simulink model "cmdvectPmsm (1)"  (R2023b)
settings: Solver=FixedStepAuto  StartTime=0.0  StopTime=0.6  FixedStep=1e-5  MaxStep=1e-6  RelTol=1e-6
undefined symbols (not defined in the file): A1, A2, B1, B2, fs, J, Ld, Lq, P, Phif
libraries: spsTriangleGeneratorLib x1
settings Model: Creator=HP  LastModifiedBy=HP
settings SolverCC: ZeroCrossAlgorithm=Adaptive
settings DebuggingCC: IgnoredZcDiagnostic=none

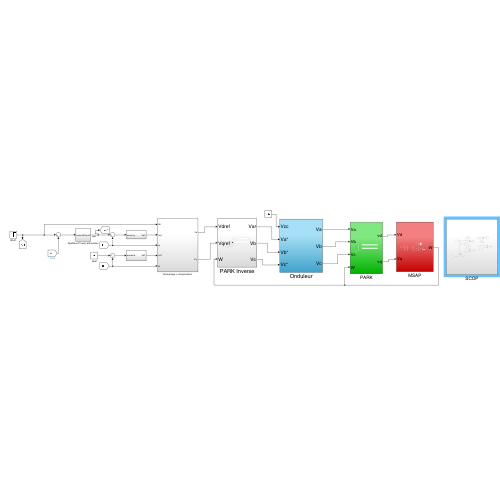
[thumbnail: Simulink's stored preview of the top-level diagram]
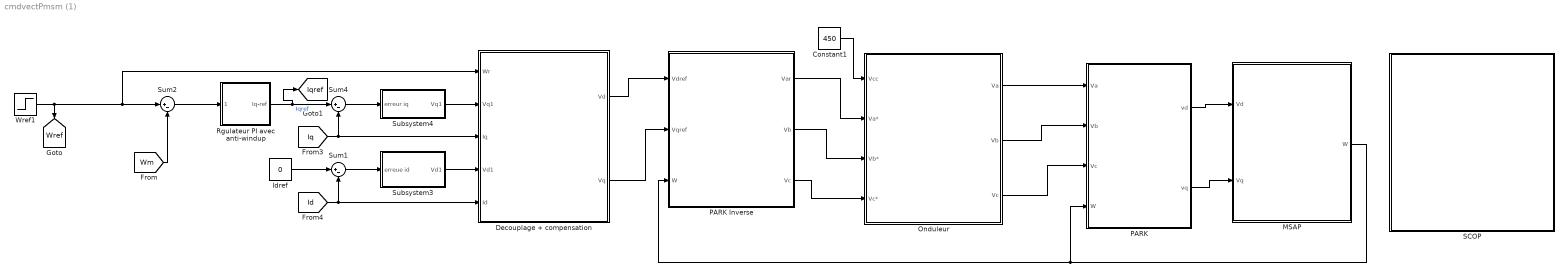
== system cmdvectPmsm (1) ==
  " Idref" : Constant  Value=0
  Constant1 : Constant  Value=450
  "Decouplage + compensation " : Subsystem
  MSAP : Subsystem
  Onduleur : Subsystem
  PARK : Subsystem
  PARK Inverse : Subsystem
  Rgulateur PI avec anti-windup : Subsystem
  SCOP : Subsystem
  Subsystem3 : Subsystem
  Subsystem4 : Subsystem
  Sum1 : Sum  Inputs=|+-
  Sum2 : Sum  Inputs=|+-
  Sum4 : Sum  Inputs=|+-
  Wref1 : Step  Time=0.3  Before=500  After=1000  SampleTime=0
  tag scope: Iqref=global, Wref=global
  wires:
  PARK/1(vd) -> MSAP/1(Vd)
  PARK/2(vq) -> MSAP/2(Vq)
  "Decouplage + compensation "/2("Vq ") -> PARK Inverse/2(Vqref)
  "Decouplage + compensation "/1(Vd) -> PARK Inverse/1(Vdref)
  Subsystem4/1(Vq1) -> "Decouplage + compensation "/2("Vq1 ")
  Subsystem3/1(Vd1) -> "Decouplage + compensation "/4("Vd1 ")
  [Iq] -> Sum4/2, "Decouplage + compensation "/3(Iq)
  Rgulateur PI avec anti-windup/1(Iq-ref) -> [Iqref], Sum4/1  "Iqref"
  Sum4/1 -> Subsystem4/1(erreur iq)
  [Id] -> "Decouplage + compensation "/5(Id), Sum1/2
  Sum1/1 -> Subsystem3/1(erreue id)
  MSAP/1(W) -> PARK Inverse/3(W), PARK/4(W)
  Wref1/1 -> [Wref], "Decouplage + compensation "/1("Wr "), Sum2/1
  " Idref"/1 -> Sum1/1
  Sum2/1 -> Rgulateur PI avec anti-windup/1(erreur Wr)
  Onduleur/1(Va) -> PARK/1(Va)
  Onduleur/2(Vb) -> PARK/2(Vb)
  Onduleur/3(Vc) -> PARK/3(Vc)
  PARK Inverse/1(Var) -> Onduleur/2(Va*)
  PARK Inverse/2(Vb) -> Onduleur/3(Vb*)
  PARK Inverse/3(Vc) -> Onduleur/4(Vc*)
  Constant1/1 -> Onduleur/1(Vcc)
  [Wm] -> Sum2/2

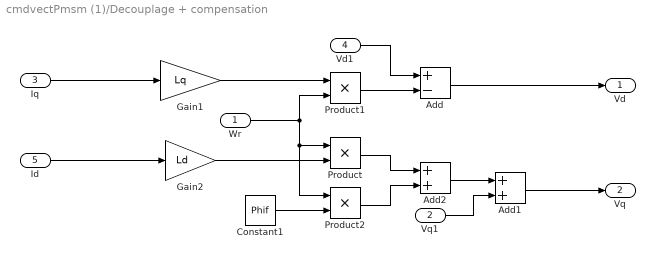
== system cmdvectPmsm (1)/Decouplage + compensation  ==
  "Wr " : Inport
  "Vq1 " : Inport  Port=2
  Iq : Inport  Port=3
  "Vd1 " : Inport  Port=4
  Id : Inport  Port=5
  Add : Sum  Inputs=+-
  Add1 : Sum
  Add2 : Sum
  Constant1 : Constant  Value=Phif
  Gain1 : Gain  Gain=Lq
  Gain2 : Gain  Gain=Ld
  Product : Product
  Product1 : Product
  Product2 : Product
  Vd : Outport
  "Vq " : Outport  Port=2
  wires:
  Iq/1 -> Gain1/1
  Add2/1 -> Add1/1
  Product1/1 -> Add/2
  Add1/1 -> "Vq "/1
  Add/1 -> Vd/1
  Product/1 -> Add2/1
  Product2/1 -> Add2/2
  Gain2/1 -> Product/2
  "Vd1 "/1 -> Add/1
  "Wr "/1 -> Product2/1, Product/1, Product1/2
  Gain1/1 -> Product1/1
  "Vq1 "/1 -> Add1/2
  Id/1 -> Gain2/1
  Constant1/1 -> Product2/2

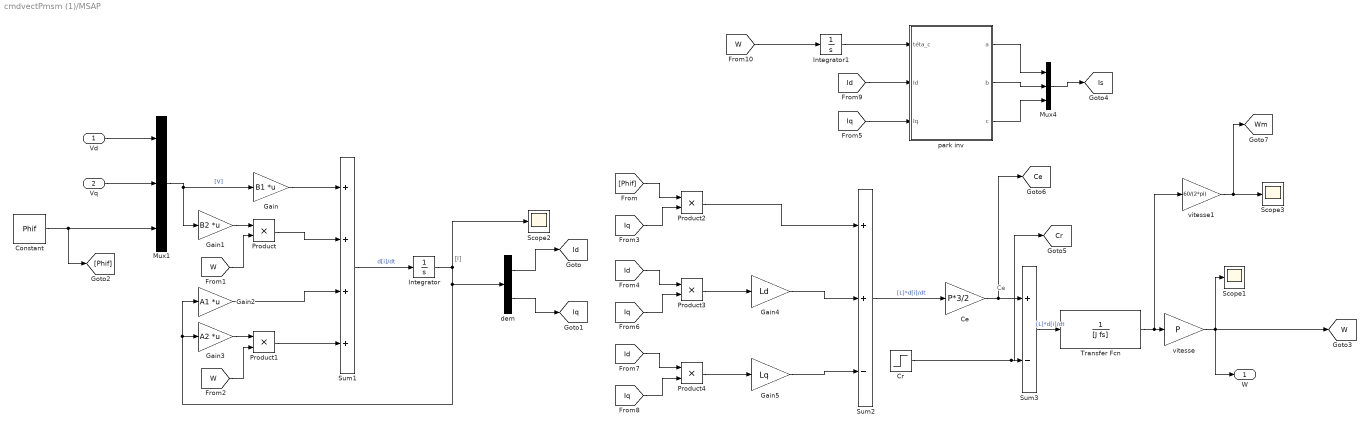
== system cmdvectPmsm (1)/MSAP ==
  note: Ce
  note: [I]
  Vd : Inport
  Vq : Inport  Port=2
  Ce : Gain  Gain=P*3/2
  Constant : Constant  Value=Phif
  Cr : Step  Time=0.3  Before=0.5  After=10  SampleTime=0
  Gain : Gain  Gain=B1  Multiplication=Matrix(K*u)
  Gain1 : Gain  Gain=B2  Multiplication=Matrix(K*u)
  Gain2 : Gain  Gain=A1  Multiplication=Matrix(K*u)
  Gain3 : Gain  Gain=A2  Multiplication=Matrix(K*u)
  Gain4 : Gain  Gain=Ld
  Gain5 : Gain  Gain=Lq
  Integrator : Integrator
  Integrator1 : Integrator
  Mux1 : Mux  Inputs=3
  Mux4 : Mux  Inputs=3
  Product{,1..4} (5 alike) : Product
  Scope1 : Scope
  Scope2 : Scope
  Scope3 : Scope
  Sum1 : Sum  Inputs=++++
  Sum2 : Sum  Inputs=++-
  Sum3 : Sum  Inputs=+-
  Transfer Fcn : TransferFcn  Denominator=[J fs]
  dem : Demux  Outputs=2
  park inv : Subsystem
  vitesse : Gain  Gain=P
  vitesse1 : Gain  Gain=60/(2*pi)
  W : Outport
  tag scope: Ce=global, Cr=global, Id=global, Iq=global, Is=global, W=global, Wm=global
  wires:
  Ce/1 -> [Ce], Sum3/1
  Constant/1 -> [Phif], Mux1/3
  Product3/1 -> Gain4/1
  Vq/1 -> Mux1/2
  Gain/1 -> Sum1/1
  Vd/1 -> Mux1/1
  [Phif] -> Product2/1
  Product2/1 -> Sum2/1
  Transfer Fcn/1 -> vitesse1/1, vitesse/1
  Gain5/1 -> Sum2/3
  Product4/1 -> Gain5/1
  dem/1 -> [Id]
  [Iq] -> Product3/2
  Gain4/1 -> Sum2/2
  [Iq] -> Product4/2
  Sum1/1 -> Integrator/1  "d[i]/dt"
  Gain3/1 -> Product1/1
  [W] -> Product/2
  dem/2 -> [Iq]
  [Id] -> Product3/1
  Integrator/1 -> dem/1, Gain3/1, Gain2/1, Scope2/1
  [Id] -> Product4/1
  Product/1 -> Sum1/2
  Sum2/1 -> Ce/1  "[L]*d[i]/dt"
  Gain1/1 -> Product/1
  Mux1/1 -> Gain1/1, Gain/1  "[V]"
  Gain2/1 -> Sum1/3
  [Iq] -> Product2/2
  Product1/1 -> Sum1/4
  [W] -> Product1/2
  Sum3/1 -> Transfer Fcn/1  "[L]*d[i]/dt"
  Cr/1 -> [Cr], Sum3/2
  [Iq] -> park inv/3(Iq)
  [Id] -> park inv/2(Id)
  park inv/3(c) -> Mux4/3
  park inv/2(b) -> Mux4/2
  park inv/1(a) -> Mux4/1
  Mux4/1 -> [Is]
  Integrator1/1 -> park inv/1(téta_c)
  [W] -> Integrator1/1
  vitesse/1 -> [W], W/1, Scope1/1
  vitesse1/1 -> [Wm], Scope3/1

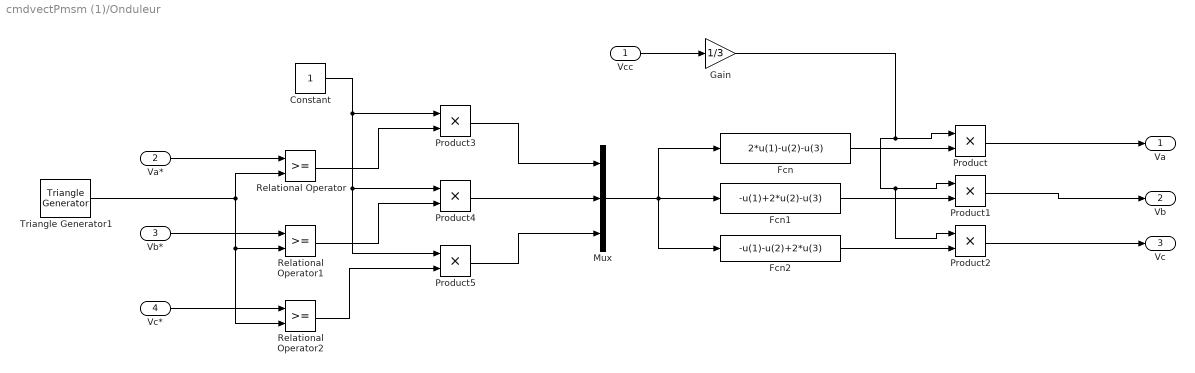
== system cmdvectPmsm (1)/Onduleur ==
  Vcc : Inport
  Va* : Inport  Port=2
  Vb* : Inport  Port=3
  Vc* : Inport  Port=4
  Constant : Constant
  Fcn : Fcn  Expr=2*u(1)-u(2)-u(3)
  Fcn1 : Fcn  Expr=-u(1)+2*u(2)-u(3)
  Fcn2 : Fcn  Expr=-u(1)-u(2)+2*u(3)
  Gain : Gain  Gain=1/3
  Mux : Mux  Inputs=3
  Product{,1..5} (6 alike) : Product
  Relational Operator : RelationalOperator  OutDataTypeStr=boolean  InputSameDT=off
  Relational Operator1 : RelationalOperator  OutDataTypeStr=boolean  InputSameDT=off
  Relational Operator2 : RelationalOperator  OutDataTypeStr=boolean  InputSameDT=off
  Triangle Generator1 : spsTriangleGeneratorLib/Triangle Generator  Freq=5e3  Phase=0  Ts=0
  Va : Outport
  Vb : Outport  Port=2
  Vc : Outport  Port=3
  wires:
  Product2/1 -> Vc/1
  Product/1 -> Va/1
  Product1/1 -> Vb/1
  Gain/1 -> Product2/1, Product1/1, Product/1
  Fcn1/1 -> Product1/2
  Vcc/1 -> Gain/1
  Mux/1 -> Fcn2/1, Fcn1/1, Fcn/1
  Product5/1 -> Mux/3
  Product3/1 -> Mux/1
  Product4/1 -> Mux/2
  Fcn/1 -> Product/2
  Fcn2/1 -> Product2/2
  Triangle Generator1/1 -> Relational Operator2/2, Relational Operator1/2, Relational Operator/2
  Va*/1 -> Relational Operator/1
  Relational Operator2/1 -> Product5/2
  Vb*/1 -> Relational Operator1/1
  Relational Operator1/1 -> Product4/2
  Constant/1 -> Product4/1, Product5/1, Product3/1
  Vc*/1 -> Relational Operator2/1
  Relational Operator/1 -> Product3/2

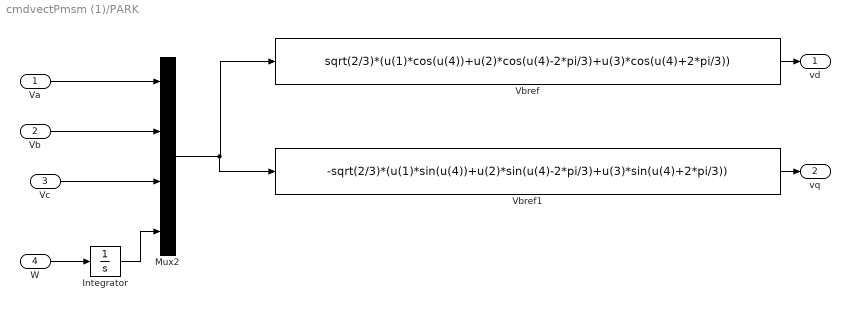
== system cmdvectPmsm (1)/PARK ==
  Va : Inport
  Vb : Inport  Port=2
  Vc : Inport  Port=3
  W : Inport  Port=4
  Integrator : Integrator
  Mux2 : Mux
  Vbref : Fcn  Expr=sqrt(2/3)*(u(1)*cos(u(4))+u(2)*cos(u(4)-2*pi/3)+u(3)*cos(u(4)+2*pi/3))
  Vbref1 : Fcn  Expr=-sqrt(2/3)*(u(1)*sin(u(4))+u(2)*sin(u(4)-2*pi/3)+u(3)*sin(u(4)+2*pi/3))
  vd : Outport
  vq : Outport  Port=2
  wires:
  Integrator/1 -> Mux2/4
  Vbref/1 -> vd/1
  Va/1 -> Mux2/1
  W/1 -> Integrator/1
  Vc/1 -> Mux2/3
  Mux2/1 -> Vbref1/1, Vbref/1
  Vbref1/1 -> vq/1
  Vb/1 -> Mux2/2

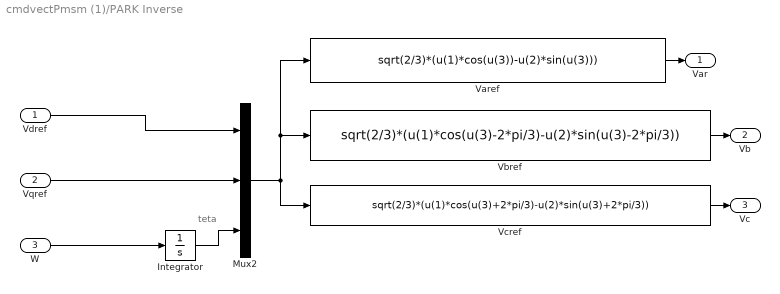
== system cmdvectPmsm (1)/PARK Inverse ==
  note: teta
  Vdref : Inport
  Vqref : Inport  Port=2
  W : Inport  Port=3
  Integrator : Integrator
  Mux2 : Mux  Inputs=3
  Varef : Fcn  Expr=sqrt(2/3)*(u(1)*cos(u(3))-u(2)*sin(u(3)))
  Vbref : Fcn  Expr=sqrt(2/3)*(u(1)*cos(u(3)-2*pi/3)-u(2)*sin(u(3)-2*pi/3))
  Vcref : Fcn  Expr=sqrt(2/3)*(u(1)*cos(u(3)+2*pi/3)-u(2)*sin(u(3)+2*pi/3))
  Var : Outport
  Vb : Outport  Port=2
  Vc : Outport  Port=3
  wires:
  W/1 -> Integrator/1
  Varef/1 -> Var/1
  Integrator/1 -> Mux2/3
  Mux2/1 -> Vcref/1, Varef/1, Vbref/1
  Vbref/1 -> Vb/1
  Vqref/1 -> Mux2/2
  Vdref/1 -> Mux2/1
  Vcref/1 -> Vc/1

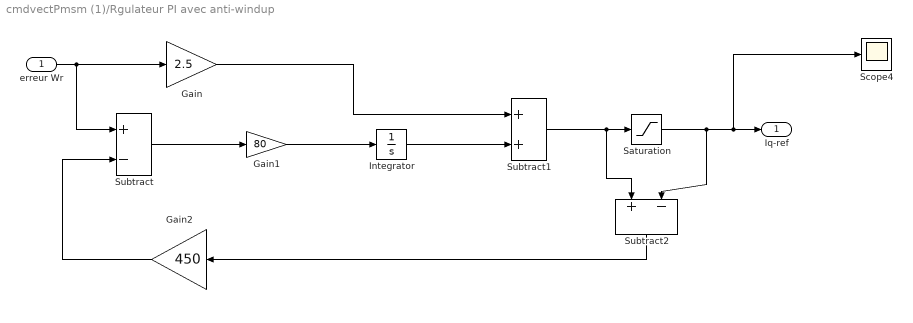
== system cmdvectPmsm (1)/Rgulateur PI avec anti-windup ==
  erreur Wr : Inport
  Gain : Gain  Gain=2.5
  Gain1 : Gain  Gain=80
  Gain2 : Gain  Gain=450
  Integrator : Integrator
  Saturation : Saturate  UpperLimit=30  LowerLimit=-30
  Scope4 : Scope
  Subtract : Sum  Inputs=+-
  Subtract1 : Sum
  Subtract2 : Sum  Inputs=+-
  Iq-ref : Outport
  wires:
  Gain1/1 -> Integrator/1
  Gain2/1 -> Subtract/2
  Saturation/1 -> Scope4/1, Iq-ref/1, Subtract2/2
  Subtract1/1 -> Subtract2/1, Saturation/1
  Gain/1 -> Subtract1/1
  Integrator/1 -> Subtract1/2
  erreur Wr/1 -> Subtract/1, Gain/1
  Subtract2/1 -> Gain2/1
  Subtract/1 -> Gain1/1

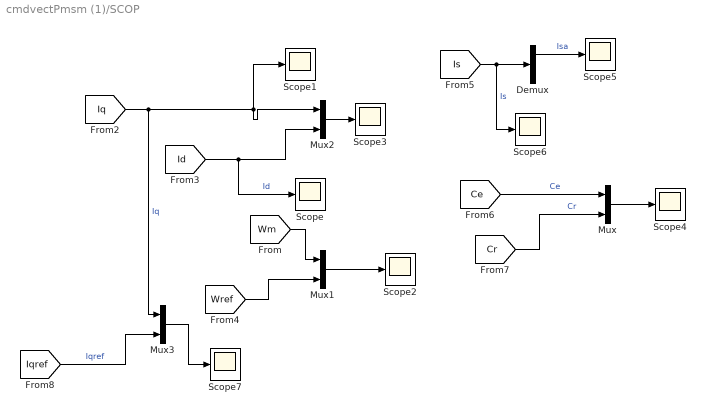
== system cmdvectPmsm (1)/SCOP ==
  Demux : Demux  Outputs=3
  Mux{,1..3} (4 alike) : Mux  Inputs=2
  Scope{,1..7} (8 alike) : Scope
  wires:
  [Id] -> Mux2/2, Scope/1  "Id"
  Mux1/1 -> Scope2/1
  [Ce] -> Mux/1  "Ce"
  Mux/1 -> Scope4/1
  [Cr] -> Mux/2  "Cr"
  [Is] -> Scope6/1, Demux/1  "Is"
  Demux/1 -> Scope5/1  "Isa"
  Mux2/1 -> Scope3/1
  [Iqref] -> Mux3/2  "Iqref"
  [Iq] -> Mux3/1, Mux2/1, Scope1/1  "Iq"
  Mux3/1 -> Scope7/1
  [Wref] -> Mux1/2
  [Wm] -> Mux1/1

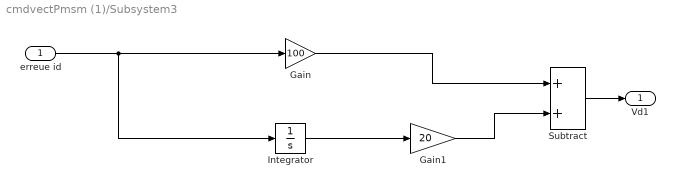
== system cmdvectPmsm (1)/Subsystem3 ==
  erreue id : Inport
  Gain : Gain  Gain=100
  Gain1 : Gain  Gain=20
  Integrator : Integrator
  Subtract : Sum
  Vd1 : Outport
  wires:
  Integrator/1 -> Gain1/1
  erreue id/1 -> Integrator/1, Gain/1
  Subtract/1 -> Vd1/1
  Gain1/1 -> Subtract/2
  Gain/1 -> Subtract/1

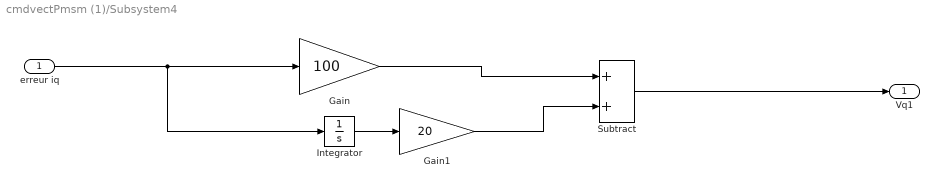
== system cmdvectPmsm (1)/Subsystem4 ==
  erreur iq : Inport
  Gain : Gain  Gain=100
  Gain1 : Gain  Gain=20
  Integrator : Integrator
  Subtract : Sum
  Vq1 : Outport
  wires:
  Integrator/1 -> Gain1/1
  erreur iq/1 -> Integrator/1, Gain/1
  Subtract/1 -> Vq1/1
  Gain1/1 -> Subtract/2
  Gain/1 -> Subtract/1

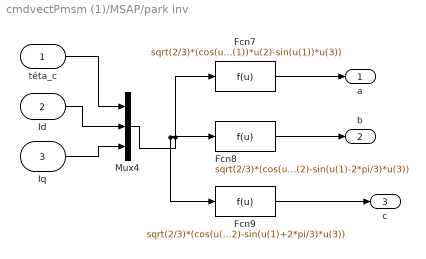
== system cmdvectPmsm (1)/MSAP/park inv ==
  téta_c : Inport
  Id : Inport  Port=2
  Iq : Inport  Port=3
  Fcn7 : Fcn  Expr=sqrt(2/3)*(cos(u(1))*u(2)-sin(u(1))*u(3))
  Fcn8 : Fcn  Expr=sqrt(2/3)*(cos(u(1)-2*pi/3)*u(2)-sin(u(1)-2*pi/3)*u(3))
  Fcn9 : Fcn  Expr=sqrt(2/3)*(cos(u(1)+2*pi/3)*u(2)-sin(u(1)+2*pi/3)*u(3))
  Mux4 : Mux  Inputs=3
  a : Outport
  b : Outport  Port=2
  c : Outport  Port=3
  wires:
  Fcn8/1 -> b/1
  Fcn9/1 -> c/1
  téta_c/1 -> Mux4/1
  Fcn7/1 -> a/1
  Iq/1 -> Mux4/3
  Mux4/1 -> Fcn7/1, Fcn8/1, Fcn9/1
  Id/1 -> Mux4/2
